simulink model "original_model_robot_hand5_servo_1"  (R2023b)
settings: Solver=VariableStepAuto  StartTime=0.0  StopTime=inf  FixedStep=0.01  MinStep=0.01  RelTol=1e-3  EnableMultiTasking=on
undefined symbols (not defined in the file or in its folder): Ts
libraries: arduinolib x15, simulink x5, dspstat3 x5, dxlSimLibrary x4
settings Model: ExtModeTrigDuration=2  Creator=Yuk  LastModifiedBy=Yuk
settings SolverCC: InitialStep=0.01  ConcurrentTasks=on  PositivePriorityOrder=on  AutoInsertRateTranBlk=on
settings OptimizationCC: BlockReduction=off  EnhancedBackFolding=on  PassReuseOutputArgsAs=Individual arguments  ZeroExternalMemoryAtStartup=off  ZeroInternalMemoryAtStartup=off  EfficientFloat2IntCast=on  MaxStackSize=64  OptimizeBlockOrder=speed  DifferentSizesBufferReuse=on  OptimizationCustomize=off  EfficientTunableParamExpr=on
settings DebuggingCC: TasksWithSamePriorityMsg=none  ParameterPrecisionLossMsg=none  ParameterTunabilityLossMsg=error  UniqueDataStoreMsg=error
settings HardwareCC: ProdBitPerInt=16  ProdBitPerPointer=16  ProdBitPerSizeT=16  ProdBitPerPtrDiffT=16  ProdLargestAtomicFloat=None  ProdWordSize=8  ProdHWDeviceType=Atmel->AVR
settings SFSimCC: MATLABDynamicMemAlloc=off
settings RTWCC: Description=Embedded Coder  SystemTargetFile=ert.tlc  HardwareBoard=Arduino Uno  TemplateMakefile=ert_default_tmf  Toolchain=Arduino AVR  BuildConfiguration=Faster Runs  CodeExecutionProfiling=on  TargetLang=C++
settings CodeAppCC: ForceParamTrailComments=on  IgnoreCustomStorageClasses=off  OperatorAnnotations=on  SimulinkDataObjDesc=on  SFDataObjDesc=on  InsertBlockDesc=on
settings ERTTargetCC: CodeInterfacePackaging=C++ class  SupportContinuousTime=on  SupportVariableSizeSignals=on  ExtModeTransport=3  ExtModeStaticAlloc=on  ExtModeAutomaticAllocSize=off  ExtModeStaticAllocSize=250  ExtModeMexFile=ext_xcp  ExtModeIntrfLevel=Level2 - Open  RootIOFormat=Structure reference

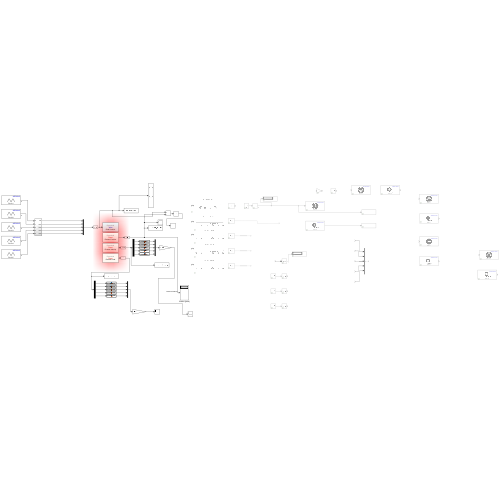
[thumbnail: Simulink's stored preview of the top-level diagram]
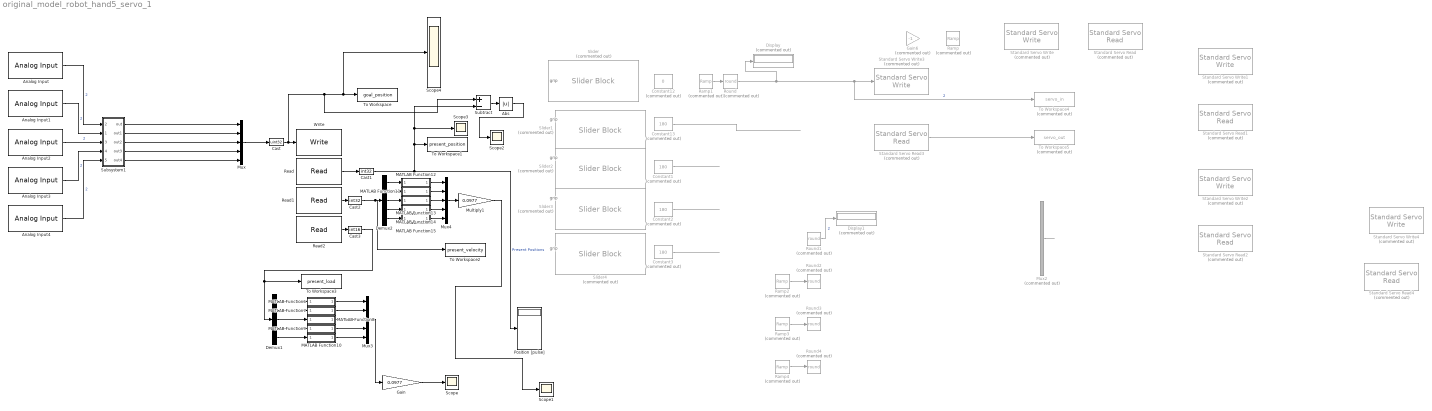
== system original_model_robot_hand5_servo_1 ==
  note: grip
  note: grip
  note: grip
  note: grip
  note: grip
  Abs : Abs  SaturateOnIntegerOverflow=off
  Analog Input : arduinolib/Analog Input  pinNumber=1  ReadResultsOnly=off  ConversionTriggerSource=Software  ExternalTriggerType=uint32( 0 )  OutputDataType=uint16  EnableConversionCompleteNotify=off  EnableOuputStatus=off  SampleTime=0.05  blockPlatform=arduino
  Analog Input1 : arduinolib/Analog Input  pinNumber=2  ReadResultsOnly=off  ConversionTriggerSource=Software  ExternalTriggerType=uint32( 0 )  OutputDataType=uint16  EnableConversionCompleteNotify=off  EnableOuputStatus=off  SampleTime=0.05  blockPlatform=arduino
  Analog Input2 : arduinolib/Analog Input  pinNumber=3  ReadResultsOnly=off  ConversionTriggerSource=Software  ExternalTriggerType=uint32( 0 )  OutputDataType=uint16  EnableConversionCompleteNotify=off  EnableOuputStatus=off  SampleTime=0.05  blockPlatform=arduino
  Analog Input3 : arduinolib/Analog Input  pinNumber=4  ReadResultsOnly=off  ConversionTriggerSource=Software  ExternalTriggerType=uint32( 0 )  OutputDataType=uint16  EnableConversionCompleteNotify=off  EnableOuputStatus=off  SampleTime=0.05  blockPlatform=arduino
  Analog Input4 : arduinolib/Analog Input  pinNumber=5  ReadResultsOnly=off  ConversionTriggerSource=Software  ExternalTriggerType=uint32( 0 )  OutputDataType=uint16  EnableConversionCompleteNotify=off  EnableOuputStatus=off  SampleTime=0.05  blockPlatform=arduino
  Cast : DataTypeConversion  OutMin=0  OutMax=2097150  OutDataTypeStr=uint32  SaturateOnIntegerOverflow=off  RndMeth=Floor
  Cast1 : DataTypeConversion  OutDataTypeStr=int32  SaturateOnIntegerOverflow=off  RndMeth=Floor
  Cast2 : DataTypeConversion  OutDataTypeStr=int32  SaturateOnIntegerOverflow=off  RndMeth=Floor
  Cast3 : DataTypeConversion  OutDataTypeStr=int16  SaturateOnIntegerOverflow=off  RndMeth=Floor
  Constant{1..3,13} (4 alike) : Constant  Commented=on  Value=180  SampleTime=0.1  LockScale=on
  Constant12 : Constant  Commented=on  Value=0  SampleTime=0.1  LockScale=on
  Demux1 : Demux  Outputs=5
  Demux2 : Demux  Outputs=5
  Display : Display  Commented=on
  Display1 : Display  Commented=on
  Gain : Gain  Gain=0.0977
  Gain6 : Gain  Commented=on  Gain=-1
  MATLAB Function10 : MATLAB Function  TreatAsAtomicUnit=on
  MATLAB Function11 : MATLAB Function  TreatAsAtomicUnit=on
  MATLAB Function12 : MATLAB Function  TreatAsAtomicUnit=on
  MATLAB Function13 : MATLAB Function  TreatAsAtomicUnit=on
  MATLAB Function14 : MATLAB Function  TreatAsAtomicUnit=on
  MATLAB Function15 : MATLAB Function  TreatAsAtomicUnit=on
  MATLAB Function6 : MATLAB Function  TreatAsAtomicUnit=on
  MATLAB Function7 : MATLAB Function  TreatAsAtomicUnit=on
  MATLAB Function8 : MATLAB Function  TreatAsAtomicUnit=on
  MATLAB Function9 : MATLAB Function  TreatAsAtomicUnit=on
  Multiply1 : Gain  Gain=0.0977  OutDataTypeStr=double
  Mux : Mux  Inputs=5
  Mux2 : Mux  Commented=on  Inputs=5
  Mux3 : Mux  Inputs=5
  Mux4 : Mux  Inputs=5
  Position [pulse] : Display
  Ramp : simulink/Sources/Ramp  Commented=on  slope=50  start=1  InitialOutput=-125
  Ramp1 : simulink/Sources/Ramp  Commented=on  slope=50  start=1  InitialOutput=70
  Ramp2 : simulink/Sources/Ramp  Commented=on  slope=50  start=10  InitialOutput=70
  Ramp3 : simulink/Sources/Ramp  Commented=on  slope=50  start=14  InitialOutput=70
  Ramp4 : simulink/Sources/Ramp  Commented=on  slope=50  start=18  InitialOutput=70
  Read : dxlSimLibrary/Read  lib_name=lib_name  port_num=port_num  protocol_version=protocol_version  ids=motor_IDs  models=motor_models  select=Present Position  Ts=Ts
  Read1 : dxlSimLibrary/Read  lib_name=lib_name  port_num=port_num  protocol_version=protocol_version  ids=motor_IDs  models=motor_models  select=Present Velocity  Ts=Ts
  Read2 : dxlSimLibrary/Read  lib_name=lib_name  port_num=port_num  protocol_version=protocol_version  ids=motor_IDs  models=motor_models  select=Present Load  Ts=Ts
  Round{,1..4} (5 alike) : Rounding  Commented=on  Operator=round
  Scope{,1..4} (5 alike) : Scope
  Slider : SliderBlock  Commented=on  ScaleMin=-125  ScaleMax=0
  Slider{1..4} (4 alike) : SliderBlock  Commented=on  ScaleMin=70  ScaleMax=180
  Standard Servo Read : arduinolib/Standard Servo Read  Commented=on  pinNumber=3  SampleTime=0.1  ServoIndex=0  blockPlatform=ARDUINO
  Standard Servo Read1 : arduinolib/Standard Servo Read  Commented=on  pinNumber=5  SampleTime=0.1  ServoIndex=0  blockPlatform=ARDUINO
  Standard Servo Read2 : arduinolib/Standard Servo Read  Commented=on  pinNumber=6  SampleTime=0.1  ServoIndex=0  blockPlatform=ARDUINO
  Standard Servo Read3 : arduinolib/Standard Servo Read  Commented=on  pinNumber=9  SampleTime=0.1  ServoIndex=0  blockPlatform=ARDUINO
  Standard Servo Read4 : arduinolib/Standard Servo Read  Commented=on  pinNumber=10  SampleTime=0.1  ServoIndex=0  blockPlatform=ARDUINO
  Standard Servo Write : arduinolib/Standard Servo Write  Commented=on  pinNumber=3  ServoIndex=0  blockPlatform=ARDUINO
  Standard Servo Write1 : arduinolib/Standard Servo Write  Commented=on  pinNumber=5  ServoIndex=0  blockPlatform=ARDUINO
  Standard Servo Write2 : arduinolib/Standard Servo Write  Commented=on  pinNumber=6  ServoIndex=0  blockPlatform=ARDUINO
  Standard Servo Write3 : arduinolib/Standard Servo Write  Commented=on  pinNumber=9  ServoIndex=0  blockPlatform=ARDUINO
  Standard Servo Write4 : arduinolib/Standard Servo Write  Commented=on  pinNumber=10  ServoIndex=0  blockPlatform=ARDUINO
  Subsystem1 : Subsystem
  Subtract : Sum  Inputs=+-
  To Workspace : ToWorkspace  VariableName=goal_position  SaveFormat=Timeseries  SampleTime=-1
  To Workspace1 : ToWorkspace  VariableName=present_position  SaveFormat=Timeseries  SampleTime=-1
  To Workspace2 : ToWorkspace  VariableName=present_velocity  SaveFormat=Timeseries  SampleTime=-1
  To Workspace3 : ToWorkspace  VariableName=present_load  SaveFormat=Timeseries  SampleTime=-1
  To Workspace4 : ToWorkspace  Commented=on  VariableName=servo_in  SaveFormat=Timeseries  SampleTime=0.05
  To Workspace5 : ToWorkspace  Commented=on  VariableName=servo_out  SaveFormat=Timeseries  SampleTime=-1
  Write : dxlSimLibrary/Write  lib_name=lib_name  port_num=port_num  protocol_version=protocol_version  ids=motor_IDs  models=motor_models  select=Goal Position  Ts=Ts
  wires:
  Read/1 -> Cast1/1
  Read2/1 -> Cast3/1
  Mux/1 -> Cast/1
  Cast1/1 -> Subtract/2, Scope3/1, To Workspace1/1, Position [pulse]/1  "Present Positions"
  Cast/1 -> Subtract/1, Scope4/1, To Workspace/1, Write/1
  Cast3/1 -> Demux1/1, To Workspace3/1
  Read1/1 -> Cast2/1
  ? -> Mux2/1
  ? -> Mux2/2
  ? -> Mux2/3
  ? -> Mux2/4
  ? -> Mux2/5
  Demux1/1 -> MATLAB Function6/1(presentLoad)
  Demux1/2 -> MATLAB Function7/1(presentLoad)
  Demux1/3 -> MATLAB Function8/1(presentLoad)
  Demux1/4 -> MATLAB Function9/1(presentLoad)
  Demux1/5 -> MATLAB Function10/1(presentLoad)
  MATLAB Function6/1(convertedLoad) -> Mux3/1
  MATLAB Function7/1(convertedLoad) -> Mux3/2
  MATLAB Function8/1(convertedLoad) -> Mux3/3
  MATLAB Function9/1(convertedLoad) -> Mux3/4
  MATLAB Function10/1(convertedLoad) -> Mux3/5
  Mux3/1 -> Gain/1
  MATLAB Function13/1(convertedVel) -> Mux4/3
  MATLAB Function14/1(convertedVel) -> Mux4/4
  MATLAB Function11/1(convertedVel) -> Mux4/2
  Demux2/4 -> MATLAB Function14/1(presentVel)
  Demux2/2 -> MATLAB Function11/1(presentVel)
  Mux4/1 -> Multiply1/1
  Demux2/5 -> MATLAB Function15/1(presentVel)
  Demux2/1 -> MATLAB Function12/1(presentVel)
  Demux2/3 -> MATLAB Function13/1(presentVel)
  MATLAB Function15/1(convertedVel) -> Mux4/5
  MATLAB Function12/1(convertedVel) -> Mux4/1
  Cast2/1 -> To Workspace2/1, Demux2/1
  Gain/1 -> Scope/1
  Mux2/1 -> ?
  Round/1 -> Standard Servo Write3/1, To Workspace4/1, Display/1  "2"
  Multiply1/1 -> Scope1/1
  Subsystem1/1(out) -> Mux/1
  Subsystem1/2(out1) -> Mux/2
  Subsystem1/3(out2) -> Mux/3
  Subsystem1/4(out3) -> Mux/4
  Subsystem1/5(out4) -> Mux/5
  Analog Input2/1 -> Subsystem1/3(3)  "2"
  Analog Input/1 -> Subsystem1/1(2)  "2"
  Analog Input4/1 -> Subsystem1/5(5)  "2"
  Analog Input1/1 -> Subsystem1/2(1)  "2"
  Analog Input3/1 -> Subsystem1/4(4)  "2"
  Subtract/1 -> Abs/1
  Abs/1 -> Scope2/1
  Ramp4/1 -> Round4/1
  ? -> Round1/1
  Ramp2/1 -> Round2/1
  Round1/1 -> Display1/1  "2"
  Ramp3/1 -> Round3/1
  Constant13/1 -> ?
  Constant1/1 -> ?
  Constant2/1 -> ?
  Constant3/1 -> ?
  Ramp1/1 -> Round/1
  Standard Servo Read3/1 -> To Workspace5/1

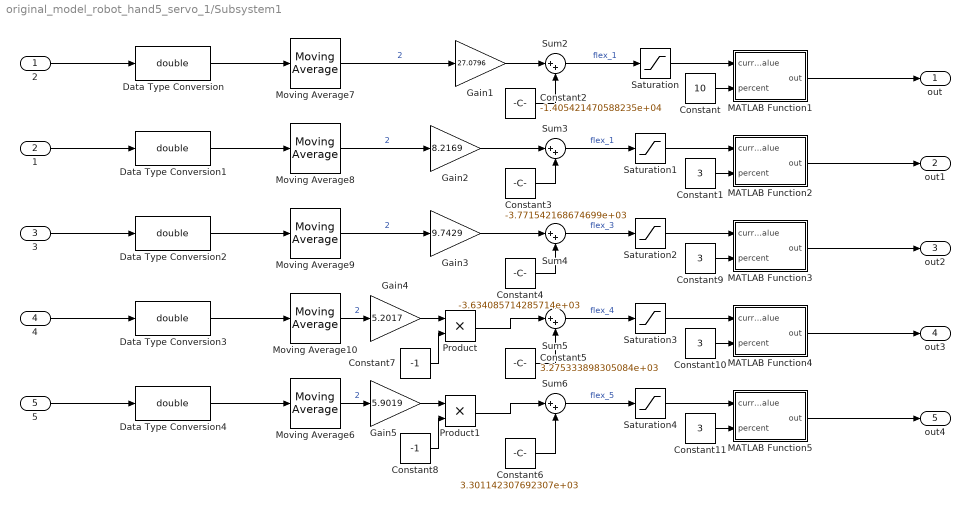
== system original_model_robot_hand5_servo_1/Subsystem1 ==
  2 : Inport
  1 : Inport  Port=2
  3 : Inport  Port=3
  4 : Inport  Port=4
  5 : Inport  Port=5
  Constant : Constant  Value=10
  Constant{1,9..11} (4 alike) : Constant  Value=3
  Constant2 : Constant  Value=-1.405421470588235e+04
  Constant3 : Constant  Value=-3.771542168674699e+03
  Constant4 : Constant  Value=-3.634085714285714e+03
  Constant5 : Constant  Value=3.275333898305084e+03
  Constant6 : Constant  Value=3.301142307692307e+03
  Constant7 : Constant  Value=-1
  Constant8 : Constant  Value=-1
  Data Type Conversion{,1..4} (5 alike) : DataTypeConversion  OutDataTypeStr=double  SaturateOnIntegerOverflow=off  RndMeth=Floor
  Gain1 : Gain  Gain=27.0796
  Gain2 : Gain  Gain=8.2169
  Gain3 : Gain  Gain=9.7429
  Gain4 : Gain  Gain=5.2017
  Gain5 : Gain  Gain=5.9019
  MATLAB Function1 : MATLAB Function  TreatAsAtomicUnit=on
  MATLAB Function2 : MATLAB Function  TreatAsAtomicUnit=on
  MATLAB Function3 : MATLAB Function  TreatAsAtomicUnit=on
  MATLAB Function4 : MATLAB Function  TreatAsAtomicUnit=on
  MATLAB Function5 : MATLAB Function  TreatAsAtomicUnit=on
  Moving Average{6..10} (5 alike) : dspstat3/Moving Average  Method=Sliding window  ForgettingFactorPort=off  SpecifyWindowLength=on  WindowLength=3  OverlapLength=2  AllowArbitraryInputLength=off  ForgettingFactor=0.9  SimulateUsing=Code generation
  Product : Product
  Product1 : Product
  Saturation : Saturate  UpperLimit=920.7  LowerLimit=0
  Saturation1 : Saturate  UpperLimit=682  LowerLimit=0
  Saturation2 : Saturate  UpperLimit=682  LowerLimit=0
  Saturation3 : Saturate  UpperLimit=1023  LowerLimit=341
  Saturation4 : Saturate  UpperLimit=1023  LowerLimit=341
  Sum{2..6} (5 alike) : Sum  Inputs=|++
  out : Outport
  out1 : Outport  Port=2
  out2 : Outport  Port=3
  out3 : Outport  Port=4
  out4 : Outport  Port=5
  wires:
  3/1 -> Data Type Conversion2/1
  5/1 -> Data Type Conversion4/1
  MATLAB Function4/1(out) -> out3/1
  MATLAB Function1/1(out) -> out/1
  MATLAB Function2/1(out) -> out1/1
  1/1 -> Data Type Conversion1/1
  Constant5/1 -> Sum5/2
  Constant9/1 -> MATLAB Function3/2(percent)
  Constant/1 -> MATLAB Function1/2(percent)
  Constant10/1 -> MATLAB Function4/2(percent)
  Sum5/1 -> Saturation3/1  "flex_4"
  Saturation/1 -> MATLAB Function1/1(currentValue)
  4/1 -> Data Type Conversion3/1
  Constant4/1 -> Sum4/2
  Moving Average6/1 -> Gain5/1  "2"
  Gain2/1 -> Sum3/1
  Constant1/1 -> MATLAB Function2/2(percent)
  MATLAB Function5/1(out) -> out4/1
  Constant8/1 -> Product1/2
  Moving Average9/1 -> Gain3/1  "2"
  Constant3/1 -> Sum3/2
  Product1/1 -> Sum6/1
  Saturation4/1 -> MATLAB Function5/1(currentValue)
  MATLAB Function3/1(out) -> out2/1
  Moving Average7/1 -> Gain1/1  "2"
  Data Type Conversion2/1 -> Moving Average9/1
  Data Type Conversion/1 -> Moving Average7/1
  Data Type Conversion4/1 -> Moving Average6/1
  Gain1/1 -> Sum2/1
  Saturation3/1 -> MATLAB Function4/1(currentValue)
  Moving Average8/1 -> Gain2/1  "2"
  Gain4/1 -> Product/1
  Constant11/1 -> MATLAB Function5/2(percent)
  Sum4/1 -> Saturation2/1  "flex_3"
  Saturation2/1 -> MATLAB Function3/1(currentValue)
  Data Type Conversion1/1 -> Moving Average8/1
  Sum3/1 -> Saturation1/1  "flex_1"
  Sum2/1 -> Saturation/1  "flex_1"
  Saturation1/1 -> MATLAB Function2/1(currentValue)
  Constant7/1 -> Product/2
  2/1 -> Data Type Conversion/1
  Constant2/1 -> Sum2/2
  Gain3/1 -> Sum4/1
  Sum6/1 -> Saturation4/1  "flex_5"
  Gain5/1 -> Product1/1
  Data Type Conversion3/1 -> Moving Average10/1
  Moving Average10/1 -> Gain4/1  "2"
  Constant6/1 -> Sum6/2
  Product/1 -> Sum5/1

== matlab function original_model_robot_hand5_servo_1/MATLAB Function14 ==
  data: presentVel input; convertedVel output
function convertedVel = convertVel(presentVel)
% Convert Dynamixel present load data from 0-2047 to -1023 to 1023
% 0-1023 remains as is, 1024-2047 is mapped to 0 to -1023

if presentVel >= 1024
    convertedVel = -(presentVel - 1024);
else
    convertedVel = presentVel;
end
end

== matlab function original_model_robot_hand5_servo_1/MATLAB Function15 ==
  data: presentVel input; convertedVel output
function convertedVel = convertVel(presentVel)
% Convert Dynamixel present load data from 0-2047 to -1023 to 1023
% 0-1023 remains as is, 1024-2047 is mapped to 0 to -1023

if presentVel >= 1024
    convertedVel = -(presentVel - 1024);
else
    convertedVel = presentVel;
end
end

== matlab function original_model_robot_hand5_servo_1/Subsystem1/MATLAB Function1 ==
  data: currentValue input; out output; percent input
function out = customDeadZone(currentValue,percent)
    % 지속적인 상태 유지를 위한 영구 변수 선언
    persistent lastValue
    if isempty(lastValue)
        lastValue = currentValue; % 최초 실행 시 초기값 설정
    end
    
    % 변화 임계값 설정
    threshold = (percent*682)/100;
    
    % 현재 값과 이전 값의 차이가 임계값보다 크면 업데이트
    if abs(currentValue - lastValue) > threshold
        lastValue = currentValue; % 값 업데이트
    end
    
    % 출력
    out = lastValue;
end

== matlab function original_model_robot_hand5_servo_1/Subsystem1/MATLAB Function3 ==
  data: currentValue input; out output; percent input
function out = customDeadZone(currentValue,percent)
    % 지속적인 상태 유지를 위한 영구 변수 선언
    persistent lastValue
    if isempty(lastValue)
        lastValue = currentValue; % 최초 실행 시 초기값 설정
    end
    
    % 변화 임계값 설정
    threshold = (percent*682)/100;
    
    % 현재 값과 이전 값의 차이가 임계값보다 크면 업데이트
    if abs(currentValue - lastValue) > threshold
        lastValue = currentValue; % 값 업데이트
    end
    
    % 출력
    out = lastValue;
end

== matlab function original_model_robot_hand5_servo_1/Subsystem1/MATLAB Function4 ==
  data: currentValue input; out output; percent input
function out = customDeadZone(currentValue,percent)
    % 지속적인 상태 유지를 위한 영구 변수 선언
    persistent lastValue
    if isempty(lastValue)
        lastValue = currentValue; % 최초 실행 시 초기값 설정
    end
    
    % 변화 임계값 설정
    threshold = (percent*682)/100;
    
    % 현재 값과 이전 값의 차이가 임계값보다 크면 업데이트
    if abs(currentValue - lastValue) > threshold
        lastValue = currentValue; % 값 업데이트
    end
    
    % 출력
    out = lastValue;
end

== matlab function original_model_robot_hand5_servo_1/Subsystem1/MATLAB Function5 ==
  data: currentValue input; out output; percent input
function out = customDeadZone(currentValue,percent)
    % 지속적인 상태 유지를 위한 영구 변수 선언
    persistent lastValue
    if isempty(lastValue)
        lastValue = currentValue; % 최초 실행 시 초기값 설정
    end
    
    % 변화 임계값 설정
    threshold = (percent*682)/100;
    
    % 현재 값과 이전 값의 차이가 임계값보다 크면 업데이트
    if abs(currentValue - lastValue) > threshold
        lastValue = currentValue; % 값 업데이트
    end
    
    % 출력
    out = lastValue;
end

== matlab function original_model_robot_hand5_servo_1/MATLAB Function6 ==
  data: presentLoad input; convertedLoad output
function convertedLoad = convertLoad(presentLoad)
% Convert Dynamixel present load data from 0-2047 to -1023 to 1023
% 0-1023 remains as is, 1024-2047 is mapped to 0 to -1023

if presentLoad >= 1024
    convertedLoad = -(presentLoad - 1024);
else
    convertedLoad = presentLoad;
end
end

== matlab function original_model_robot_hand5_servo_1/MATLAB Function7 ==
  data: presentLoad input; convertedLoad output
function convertedLoad = convertLoad(presentLoad)
% Convert Dynamixel present load data from 0-2047 to -1023 to 1023
% 0-1023 remains as is, 1024-2047 is mapped to 0 to -1023

if presentLoad >= 1024
    convertedLoad = -(presentLoad - 1024);
else
    convertedLoad = presentLoad;
end
end

== matlab function original_model_robot_hand5_servo_1/MATLAB Function8 ==
  data: presentLoad input; convertedLoad output
function convertedLoad = convertLoad(presentLoad)
% Convert Dynamixel present load data from 0-2047 to -1023 to 1023
% 0-1023 remains as is, 1024-2047 is mapped to 0 to -1023

if presentLoad >= 1024
    convertedLoad = -(presentLoad - 1024);
else
    convertedLoad = presentLoad;
end
end

== matlab function original_model_robot_hand5_servo_1/MATLAB Function9 ==
  data: presentLoad input; convertedLoad output
function convertedLoad = convertLoad(presentLoad)
% Convert Dynamixel present load data from 0-2047 to -1023 to 1023
% 0-1023 remains as is, 1024-2047 is mapped to 0 to -1023

if presentLoad >= 1024
    convertedLoad = -(presentLoad - 1024);
else
    convertedLoad = presentLoad;
end
end

== matlab function original_model_robot_hand5_servo_1/MATLAB Function10 ==
  data: presentLoad input; convertedLoad output
function convertedLoad = convertLoad(presentLoad)
% Convert Dynamixel present load data from 0-2047 to -1023 to 1023
% 0-1023 remains as is, 1024-2047 is mapped to 0 to -1023

if presentLoad >= 1024
    convertedLoad = -(presentLoad - 1024);
else
    convertedLoad = presentLoad;
end
end

== matlab function original_model_robot_hand5_servo_1/Subsystem1/MATLAB Function2 ==
  data: currentValue input; out output; percent input
function out = customDeadZone(currentValue,percent)
    % 지속적인 상태 유지를 위한 영구 변수 선언
    persistent lastValue
    if isempty(lastValue)
        lastValue = currentValue; % 최초 실행 시 초기값 설정
    end
    
    % 변화 임계값 설정
    threshold = (percent*682)/100;
    
    % 현재 값과 이전 값의 차이가 임계값보다 크면 업데이트
    if abs(currentValue - lastValue) > threshold
        lastValue = currentValue; % 값 업데이트
    end
    
    % 출력
    out = lastValue;
end

== matlab function original_model_robot_hand5_servo_1/MATLAB Function11 ==
  data: presentVel input; convertedVel output
function convertedVel = convertVel(presentVel)
% Convert Dynamixel present load data from 0-2047 to -1023 to 1023
% 0-1023 remains as is, 1024-2047 is mapped to 0 to -1023

if presentVel >= 1024
    convertedVel = -(presentVel - 1024);
else
    convertedVel = presentVel;
end
end

== matlab function original_model_robot_hand5_servo_1/MATLAB Function12 ==
  data: presentVel input; convertedVel output
function convertedVel = convertVel(presentVel)
% Convert Dynamixel present load data from 0-2047 to -1023 to 1023
% 0-1023 remains as is, 1024-2047 is mapped to 0 to -1023

if presentVel >= 1024
    convertedVel = -(presentVel - 1024);
else
    convertedVel = presentVel;
end
end

== matlab function original_model_robot_hand5_servo_1/MATLAB Function13 ==
  data: presentVel input; convertedVel output
function convertedVel = convertVel(presentVel)
% Convert Dynamixel present load data from 0-2047 to -1023 to 1023
% 0-1023 remains as is, 1024-2047 is mapped to 0 to -1023

if presentVel >= 1024
    convertedVel = -(presentVel - 1024);
else
    convertedVel = presentVel;
end
end
